simulink model "DHIYA_Phase3"  (R2026a)
settings: Solver=FixedStepDiscrete  StopTime=24  FixedStep=0.016666666666666666
InitFcn:
  | DHIYA_Load_Data
settings Model: Creator=PCD  LastModifiedBy=PCD

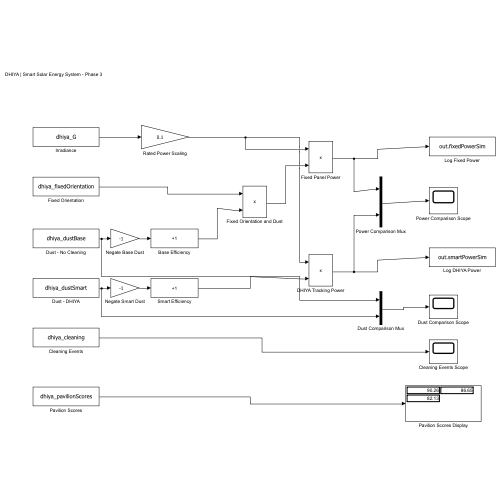
[thumbnail: Simulink's stored preview of the top-level diagram]
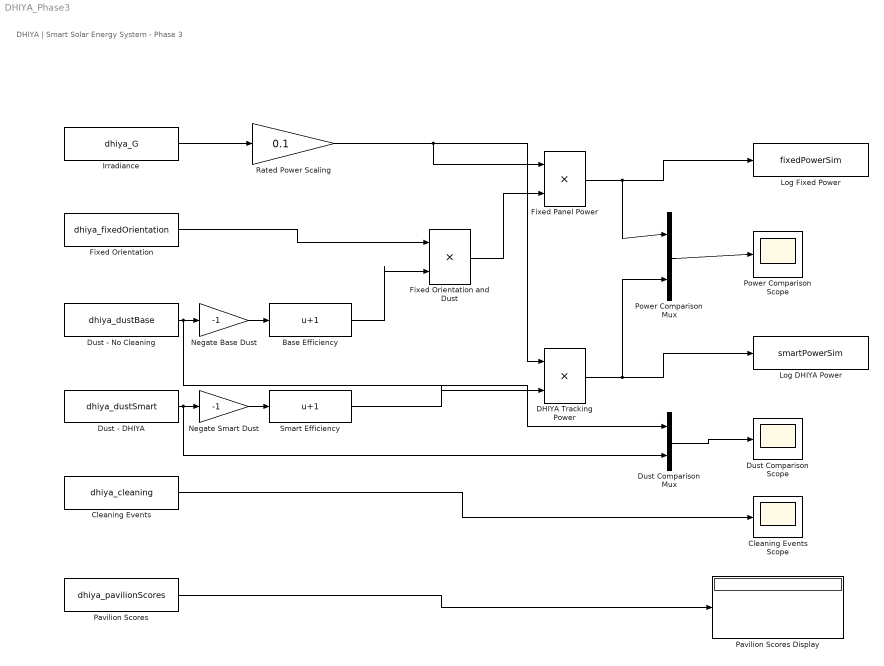
== system DHIYA_Phase3 ==
  note: DHIYA | Smart Solar Energy System - Phase 3
  Base Efficiency : Bias  Bias=1  SaturateOnIntegerOverflow=off
  Cleaning Events : FromWorkspace  VariableName=dhiya_cleaning
  Cleaning Events Scope : Scope
      settings: ActiveDisplayYMinimum=-1  ActiveDisplayYMaximum=1
  DHIYA Tracking Power : Product
  Dust - DHIYA : FromWorkspace  VariableName=dhiya_dustSmart
  Dust - No Cleaning : FromWorkspace  VariableName=dhiya_dustBase
  Dust Comparison Mux : Mux  Inputs=2
  Dust Comparison Scope : Scope
      settings: ActiveDisplayYMinimum=-1  ActiveDisplayYMaximum=1
  Fixed Orientation : FromWorkspace  VariableName=dhiya_fixedOrientation
  Fixed Orientation and Dust : Product
  Fixed Panel Power : Product
  Irradiance : FromWorkspace  VariableName=dhiya_G
  Log DHIYA Power : ToWorkspace  VariableName=smartPowerSim  SaveFormat=Timeseries  SampleTime=-1
  Log Fixed Power : ToWorkspace  VariableName=fixedPowerSim  SaveFormat=Timeseries  SampleTime=-1
  Negate Base Dust : Gain  Gain=-1
  Negate Smart Dust : Gain  Gain=-1
  Pavilion Scores : FromWorkspace  VariableName=dhiya_pavilionScores
  Pavilion Scores Display : Display
  Power Comparison Mux : Mux  Inputs=2
  Power Comparison Scope : Scope
  Rated Power Scaling : Gain  Gain=0.1
  Smart Efficiency : Bias  Bias=1  SaturateOnIntegerOverflow=off
  wires:
  Irradiance/1 -> Rated Power Scaling/1
  Dust - No Cleaning/1 -> Negate Base Dust/1, Dust Comparison Mux/1
  Negate Base Dust/1 -> Base Efficiency/1
  Dust - DHIYA/1 -> Negate Smart Dust/1, Dust Comparison Mux/2
  Negate Smart Dust/1 -> Smart Efficiency/1
  Fixed Orientation/1 -> Fixed Orientation and Dust/1
  Base Efficiency/1 -> Fixed Orientation and Dust/2
  Rated Power Scaling/1 -> Fixed Panel Power/1, DHIYA Tracking Power/1
  Fixed Orientation and Dust/1 -> Fixed Panel Power/2
  Smart Efficiency/1 -> DHIYA Tracking Power/2
  Fixed Panel Power/1 -> Power Comparison Mux/1, Log Fixed Power/1
  DHIYA Tracking Power/1 -> Power Comparison Mux/2, Log DHIYA Power/1
  Power Comparison Mux/1 -> Power Comparison Scope/1
  Dust Comparison Mux/1 -> Dust Comparison Scope/1
  Cleaning Events/1 -> Cleaning Events Scope/1
  Pavilion Scores/1 -> Pavilion Scores Display/1
